simulink subsystem "Odometria"  (R2022b)
settings: Solver=VariableStepAuto  StartTime=0.0  StopTime=10.0  RelTol=1e-3
settings Model: Creator=miriamfreiriasanjuan  LastModifiedBy=miriamfreiriasanjuan

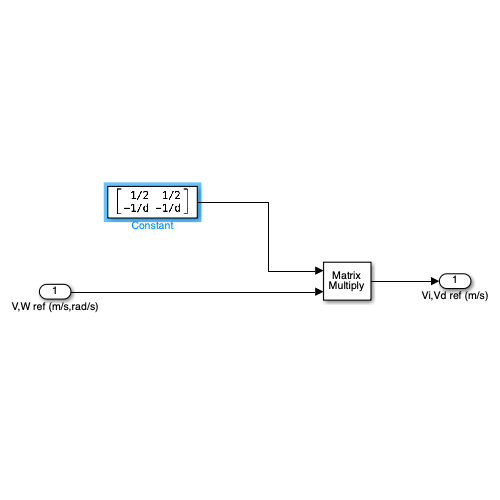
[thumbnail: Simulink's stored preview of the top-level diagram]
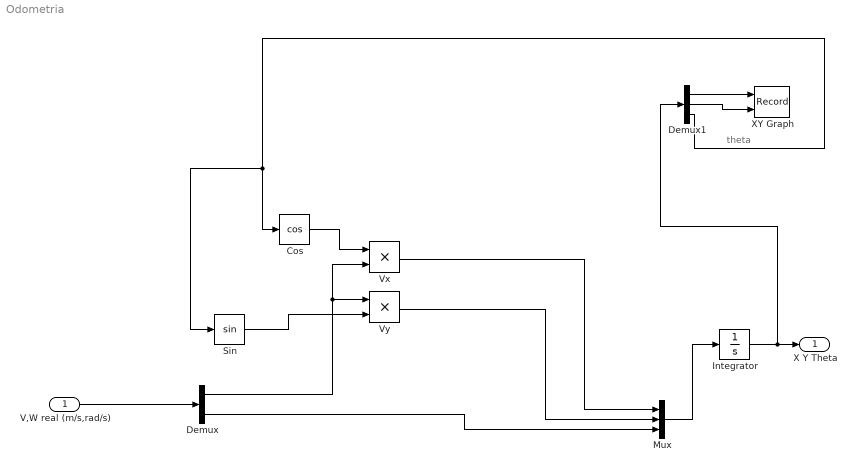
== system Odometria ==
  note: theta
  V,W real (m/s,rad/s) : Inport  OutDataTypeStr=double  PortDimensions=2
  Cos : Trigonometry  Operator=cos
  Demux : Demux  Outputs=2
  Demux1 : Demux  Outputs=3
  Integrator : Integrator
  Mux : Mux  Inputs=3
  Sin : Trigonometry
  Vx : Product
  Vy : Product
  XY Graph : Record  FileSettingsInternal="{\"entries\":[{\"content\":{\"excelSettings\":{\"content\":{},\"type\":\"Streamout.ExcelSettings\"}},\"type\":\"Streamout.FileSettingStorage\",\"uuid\":\"\"}],\"packageUris\":[\"http:\\/\\/schema.mathworks.com\\/mf0\\/streamout_blocks\\/R2020a\"],\"version\":\"1.0\"}"  Layout=[1 1]  SignalsInternal="{\"entries\":[{\"content\":{\"signals\":[{\"content\":{\"blockPath\":[],\"channel\":[],\"dimensions\":[1],\"domain\":\"\",\"lineColor\":\"#a2142f\",\"plots\":[1],\"port\":1,\"sid\":[],\"signalID\":32,\"signalName\":\"XY Graph:1\"},\"type\":\"RecordBlkView.Signal\",\"uuid\":\"\"},{\"content\":{\"blockPath\":[],\"channel\":[],\"dimensions\":[1],\"domain\":\"\",\"lineColor\":\"#139fff\",\"plots\":[1],\"port\":2,\"sid\":[],\"signalID\":35,\"signalName\":\"XY Graph:2\"},\"type\":\"RecordBlkView.Signal\",\"uuid\":\"\"}]},\"type\":\"RecordBlkView.InputSignals\",\"uuid\":\"\"}],\"packageUris\":[\"http:\\/\\/schema.mathworks.com\\/mf0\\/streamout_blocks\\/R2020a\"],\"version\":\"1.0\"}"  VisualizationBindings="{\"xyplotplugin\":{\"info\":[{\"series\":[{\"bindingParametersList\":[{\"parameter\":\"X-Axis\",\"signalID\":32,\"signalName\":\"XY Graph:1\"},{\"parameter\":\"Y-Axis\",\"signalID\":35,\"signalName\":\"XY Graph:2\"}],\"seriesID\":38784}],\"subplotID\":1}]}}"  CompatibilityTag=XY
  X Y Theta : Outport
  wires:
  V,W real (m/s,rad/s)/1 -> Demux/1
  Mux/1 -> Integrator/1
  Integrator/1 -> X Y Theta/1, Demux1/1
  Demux/2 -> Mux/3
  Vy/1 -> Mux/2
  Vx/1 -> Mux/1
  Demux/1 -> Vy/1, Vx/2
  Cos/1 -> Vx/1
  Sin/1 -> Vy/2
  Demux1/1 -> XY Graph/1
  Demux1/2 -> XY Graph/2
  Demux1/3 -> Cos/1, Sin/1
